simulink model "LabExam42"  (R2024b)
settings: Solver=VariableStepAuto  StartTime=0.0  StopTime=0.02  RelTol=1e-3
undefined symbols (not defined in the file): Angle, Magnitude
libraries: spsVoltageMeasurementLib x6, spsCurrentMeasurementLib x4, spsSeriesRLCBranchLib x4, spsACVoltageSourceLib x2, spsLinearTransformerLib x2, spspowerguiLib x2, spsRMSLib x1
settings Model: Creator=Siddharth  LastModifiedBy=HP

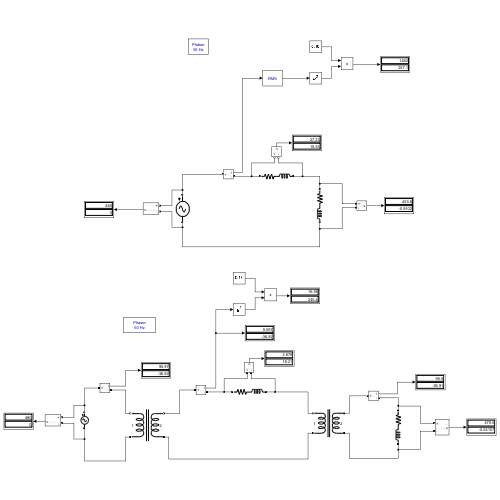
[thumbnail: Simulink's stored preview of the top-level diagram]
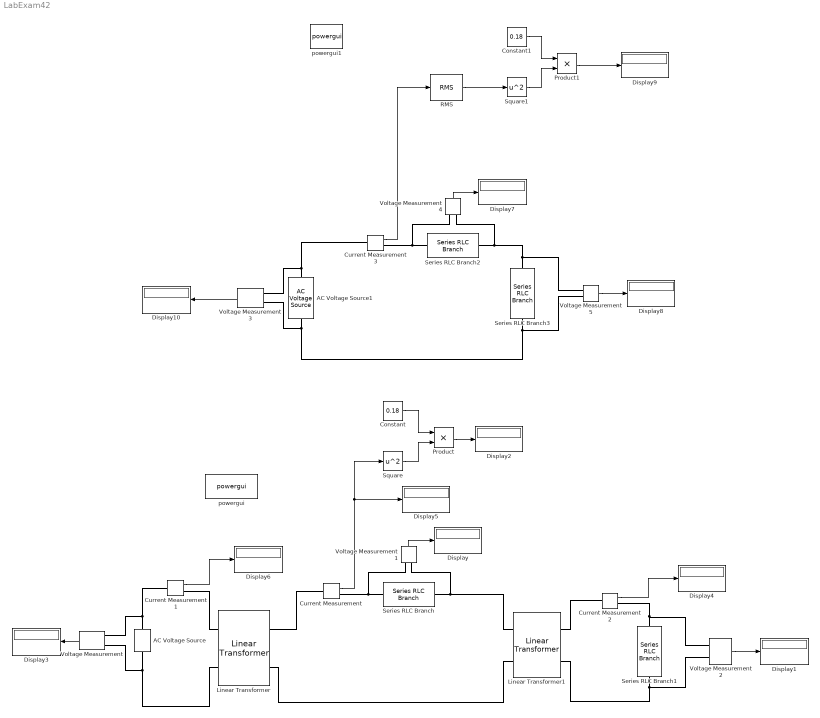
== system LabExam42 ==
  AC Voltage Source : spsACVoltageSourceLib/AC Voltage Source  Amplitude=480  Phase=0  Frequency=50  SampleTime=0  Measurements=None  BusType=swing  Pref=10e3  Qref=0  Qmin=-inf  Qmax=+inf
  AC Voltage Source1 : spsACVoltageSourceLib/AC Voltage Source  Amplitude=480  Phase=0  Frequency=50  SampleTime=0  Measurements=None  BusType=swing  Pref=10e3  Qref=0  Qmin=-inf  Qmax=+inf
  Constant : Constant  Value=0.18
  Constant1 : Constant  Value=0.18
  Current Measurement{,1..3} (4 alike) : spsCurrentMeasurementLib/Current Measurement  PhasorSimulation=on  OutputType=Magnitude-Angle  PSBequivalent=0
  Display{,1..10} (11 alike) : Display
  Linear Transformer : spsLinearTransformerLib/Linear Transformer  UNITS=SI  NominalPower=[ 250e6 50 ]  winding1=[480 0.000001 0.000001]  winding2=[4800 0.000001 0.000001]  ThreeWindings=off  winding3=[3.15e+05 0.7938 0.10107]  RmLm=[1.0804e+06 2866]  Measurements=None  DataType=on
  Linear Transformer1 : spsLinearTransformerLib/Linear Transformer  UNITS=SI  NominalPower=[ 250e6 50 ]  winding1=[4800 0.00001 0.00001]  winding2=[480 0.000001 0.00001]  ThreeWindings=off  winding3=[3.15e+05 0.7938 0.10107]  RmLm=[1.0804e+06 2866]  Measurements=None  DataType=on
  Product : Product
  Product1 : Product
  RMS : spsRMSLib/RMS  TrueRMS=on  Freq=60  RMSInit=120  Ts=0
  Series RLC Branch : spsSeriesRLCBranchLib/Series RLC Branch  LConnTagsString=__new0  RConnTagsString=__new0  BranchType=RL  Resistance=0.18  Inductance=0.24/(2*pi*50)  SetiL0=off  InitialCurrent=0  Capacitance=0  Setx0=off  InitialVoltage=0  Measurements=None
  Series RLC Branch1 : spsSeriesRLCBranchLib/Series RLC Branch  LConnTagsString=__new0  RConnTagsString=__new0  BranchType=RL  Resistance=4  Inductance=3/(2*pi*50)  SetiL0=off  InitialCurrent=0  Capacitance=0  Setx0=off  InitialVoltage=0  Measurements=None
  Series RLC Branch2 : spsSeriesRLCBranchLib/Series RLC Branch  LConnTagsString=__new0  RConnTagsString=__new0  BranchType=RL  Resistance=0.18  Inductance=0.0007643312  SetiL0=off  InitialCurrent=0  Capacitance=0  Setx0=off  InitialVoltage=0  Measurements=None
  Series RLC Branch3 : spsSeriesRLCBranchLib/Series RLC Branch  LConnTagsString=__new0  RConnTagsString=__new0  BranchType=RL  Resistance=4  Inductance=0.0095541401  SetiL0=off  InitialCurrent=0  Capacitance=0  Setx0=off  InitialVoltage=0  Measurements=None
  Square : Math  Operator=square
  Square1 : Math  Operator=square
  Voltage Measurement{,1..5} (6 alike) : spsVoltageMeasurementLib/Voltage Measurement  PhasorSimulation=on  OutputType=Magnitude-Angle  PSBequivalent=0
  powergui : spspowerguiLib/powergui  Priority=1  SimulationMode=Phasor  SampleTime=50e-6  frequency=50  Iterations=50  frequencyindice=50  Pbase=100e6  ErrMax=1e-4  UnitsV=kV  UnitsW=MW  buscounter=0  FunctionMessages=off  echomessages=off  EnableUseOfTLC=off  CurrentSourceSwitches=off  DisableSnubberDevices=off  DisableRonSwitches=off  DisableVfSwitches=off  DisplayEquations=off  AutomaticDiscreteSolvers=off  SolverType=Tustin/Backward Euler (TBE)  Interpol=off  ExternalGateDelay=off  methode=off  Ts=100  x0status=blocks  SPID=on  SwTol=0  HookPort=off  NonlinearTolerance=1e-4  nMaxIteration=100  ContinueOnMaxIteration=off  RestoreLinks=warning  ResistiveCurrentMeasurement=off  Frange=[0:2:500]  Ylog=off  Xlog=on  ShowGrid=off  save=off  variable=ZData  structure=0  ZoomFFT=off  StartTime=0.0  cycles=1  DisplayStyle=1  fundamental=60  FreqAxis=off  MaxFrequency=1000  frequencyindicesteady=1  RmsSteady=1  display=off
  powergui1 : spspowerguiLib/powergui  Priority=1  SimulationMode=Phasor  SampleTime=50e-6  frequency=50  Iterations=50  frequencyindice=50  Pbase=100e6  ErrMax=1e-4  UnitsV=kV  UnitsW=MW  buscounter=0  FunctionMessages=off  echomessages=off  EnableUseOfTLC=off  CurrentSourceSwitches=off  DisableSnubberDevices=off  DisableRonSwitches=off  DisableVfSwitches=off  DisplayEquations=off  AutomaticDiscreteSolvers=off  SolverType=Tustin/Backward Euler (TBE)  Interpol=off  ExternalGateDelay=off  methode=off  Ts=100  x0status=blocks  SPID=on  SwTol=0  HookPort=off  NonlinearTolerance=1e-4  nMaxIteration=100  ContinueOnMaxIteration=off  RestoreLinks=warning  ResistiveCurrentMeasurement=off  Frange=[0:2:500]  Ylog=off  Xlog=on  ShowGrid=off  save=off  variable=ZData  structure=0  ZoomFFT=off  StartTime=0.0  cycles=1  DisplayStyle=1  fundamental=60  FreqAxis=off  MaxFrequency=1000  frequencyindicesteady=1  RmsSteady=1  display=off
  wires:
  Constant/1 -> Product/1
  Voltage Measurement2/1 -> Display1/1
  Voltage Measurement/1 -> Display3/1
  Product/1 -> Display2/1
  Square/1 -> Product/2
  Voltage Measurement1/1 -> Display/1
  Current Measurement2/1 -> Display4/1
  Current Measurement1/1 -> Display6/1
  Current Measurement/1 -> Square/1, Display5/1
  Voltage Measurement3/1 -> Display10/1
  Product1/1 -> Display9/1
  Voltage Measurement5/1 -> Display8/1
  Current Measurement3/1 -> RMS/1
  RMS/1 -> Square1/1
  Constant1/1 -> Product1/1
  Square1/1 -> Product1/2
  Voltage Measurement4/1 -> Display7/1
  connections:
  Linear Transformer/LConn2 -- AC Voltage Source/LConn1 -- Voltage Measurement/LConn2
  Series RLC Branch/LConn1 -- Current Measurement/RConn1 -- Voltage Measurement1/LConn1
  Series RLC Branch/RConn1 -- Linear Transformer1/LConn1 -- Voltage Measurement1/LConn2
  Voltage Measurement/LConn1 -- AC Voltage Source/RConn1 -- Current Measurement1/LConn1
  Current Measurement1/RConn1 -- Linear Transformer/LConn1
  Current Measurement/LConn1 -- Linear Transformer/RConn1
  Linear Transformer/RConn2 -- Linear Transformer1/LConn2
  Linear Transformer1/RConn1 -- Current Measurement2/LConn1
  Current Measurement2/RConn1 -- Voltage Measurement2/LConn1 -- Series RLC Branch1/LConn1
  Linear Transformer1/RConn2 -- Voltage Measurement2/LConn2 -- Series RLC Branch1/RConn1
  Series RLC Branch3/LConn1 -- Series RLC Branch2/RConn1 -- Voltage Measurement4/LConn2 -- Voltage Measurement5/LConn1
  Series RLC Branch3/RConn1 -- AC Voltage Source1/LConn1 -- Voltage Measurement3/LConn2 -- Voltage Measurement5/LConn2
  Series RLC Branch2/LConn1 -- Current Measurement3/RConn1 -- Voltage Measurement4/LConn1
  AC Voltage Source1/RConn1 -- Current Measurement3/LConn1 -- Voltage Measurement3/LConn1
